simulink model "Copy_of_sistema"  (R2026b)
settings: Solver=VariableStepAuto  MaxStep=1e-3
libraries: slpidlib x1
settings Model: LastModifiedBy=Emiliano
settings DataIOCC: DSMLogging=off  ReturnWorkspaceOutputs=off  SaveOutput=off  SignalLogging=off  TimeSaveName=t
settings DebuggingCC: AlgebraicLoopMsg=none  ArtificialAlgebraicLoopMsg=none  MaxConsecutiveZCsMsg=none

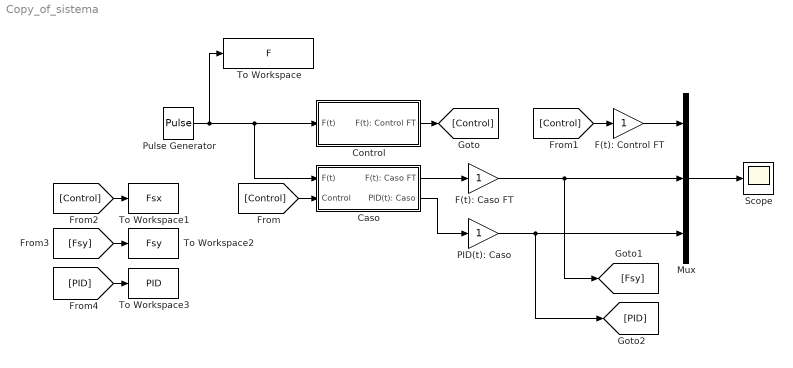
== system Copy_of_sistema ==
  Caso : Subsystem
  Control : Subsystem
  F(t): Caso FT : Gain
  F(t): Control FT : Gain
  Mux : Mux  Inputs=3
  PID(t): Caso : Gain
  Pulse Generator : DiscretePulseGenerator  PulseType=Time based  Period=10  PulseWidth=10  PhaseDelay=1
  Scope : Scope
      settings: ActiveDisplayYMinimum=-0.2  ActiveDisplayYMaximum=1
  To Workspace : ToWorkspace  VariableName=F  SampleTime=-1
  To Workspace1 : ToWorkspace  VariableName=Fsx  SampleTime=-1
  To Workspace2 : ToWorkspace  VariableName=Fsy  SampleTime=-1
  To Workspace3 : ToWorkspace  VariableName=PID  SampleTime=-1
  wires:
  Pulse Generator/1 -> To Workspace/1, Caso/1(F(t)), Control/1(F(t))
  Mux/1 -> Scope/1
  Control/1(F(t): Control FT) -> [Control]
  [Control] -> Caso/2(Control)
  Caso/1(F(t): Caso FT) -> F(t): Caso FT/1
  F(t): Caso FT/1 -> [Fsy], Mux/2
  Caso/2(PID(t): Caso) -> PID(t): Caso/1
  PID(t): Caso/1 -> [PID], Mux/3
  [Control] -> F(t): Control FT/1
  F(t): Control FT/1 -> Mux/1
  [Control] -> To Workspace1/1
  [Fsy] -> To Workspace2/1
  [PID] -> To Workspace3/1

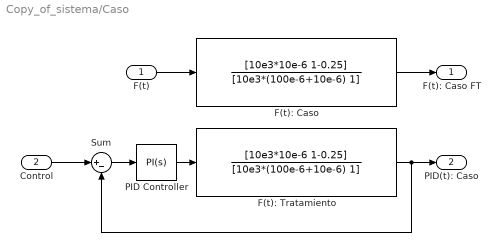
== system Copy_of_sistema/Caso ==
  F(t) : Inport
  Control : Inport  Port=2
  F(t): Caso : TransferFcn  Numerator=[10e3*10e-6 1-0.25]  Denominator=[10e3*(100e-6+10e-6) 1]
  F(t): Tratamiento : TransferFcn  Numerator=[10e3*10e-6 1-0.25]  Denominator=[10e3*(100e-6+10e-6) 1]
  PID Controller : slpidlib/PID Controller  Controller=PI  Form=Parallel  TimeDomain=Continuous-time  UseExternalTs=off  SampleTime=-1  IntegratorMethod=Forward Euler  FilterMethod=Forward Euler  ControllerParametersSource=internal  P=0.019136  I=47422.9366  UseKiTs=off  D=0  UseExternalDerivativeSource=off  N=100  UseFilter=on  TunerSelectOption=Transfer Function Based (PID Tuner App)  InitialConditionSource=internal  InitialConditionForIntegrator=0  InitialConditionForFilter=0  DifferentiatorICPrevScaledInput=0  ExternalReset=none  TrackingMode=off  Kt=1  LimitOutput=off  SatLimitsSource=internal  UpperSaturationLimit=inf  LowerSaturationLimit=-inf  LinearizeAsGain=on  AntiWindupMode=none  Kb=1  LimitIntegrator=off  UpperIntegratorSaturationLimit=inf  LowerIntegratorSaturationLimit=-inf  POutMin=[]  POutMax=[]  IOutMin=[]  IOutMax=[]  DOutMin=[]  DOutMax=[]  NOutMin=[]  NOutMax=[]  SumOutMin=[]  SumOutMax=[]  SaturationOutMin=[]  SaturationOutMax=[]  PParamMin=[]  PParamMax=[]  IParamMin=[]  IParamMax=[]  DParamMin=[]  DParamMax=[]  NParamMin=[]  NParamMax=[]  KbParamMin=[]  KbParamMax=[]  KtParamMin=[]  KtParamMax=[]  KbOutMin=[]  KbOutMax=[]  KtOutMin=[]  KtOutMax=[]  IntegratorOutMin=[]  IntegratorOutMax=[]  FilterOutMin=[]  FilterOutMax=[]  SumI1OutMin=[]  SumI1OutMax=[]  SumI2OutMin=[]  SumI2OutMax=[]  SumI3OutMin=[]  SumI3OutMax=[]  SumI4OutMin=[]  SumI4OutMax=[]  SumDOutMin=[]  SumDOutMax=[]  DifferentiatorOutMin=[]  DifferentiatorOutMax=[]  FilterDiffOutCoefMin=[]  FilterDiffOutCoefMax=[]  ReciprocalOutMin=[]  ReciprocalOutMax=[]  SumDenOutMin=[]  SumDenOutMax=[]  SumNumOutMin=[]  SumNumOutMax=[]  DivideOutMin=[]  DivideOutMax=[]  UdiffTsProdOutMin=[]  UdiffTsProdOutMax=[]  NTsProdOutMin=[]  NTsProdOutMax=[]  UintegralTsProdOutMin=[]  UintegralTsProdOutMax=[]  UngainTsProdOutMin=[]  UngainTsProdOutMax=[]  ClampingZeroOutDataTypeStr=Inherit: Inherit via back propagation  ClampingZeroOutMin=[]  ClampingZeroOutMax=[]  FilterDenConstantOutDataTypeStr=Inherit: Inherit via back propagation  FilterDenConstantOutMin=[]  FilterDenConstantOutMax=[]  PCopyOutDataTypeStr=Inherit: Inherit via back propagation  PCopyOutMin=[]  PCopyOutMax=[]  NCopyOutDataTypeStr=Inherit: Inherit via back propagation  NCopyOutMin=[]  NCopyOutMax=[]  IntegratorContinuousStateAttributes=''  IntegratorStateMustResolveToSignalObject=off  IntegratorRTWStateStorageClass=Auto  FilterContinuousStateAttributes=''  FilterStateMustResolveToSignalObject=off  FilterRTWStateStorageClass=Auto  ParallelPVariant=InternalParameters  IdealPVariant=Disabled  IVariant=InternalParameters  DVariant=Disabled  IntegratorVariant=Continuous  SatVariant=Disabled  AWVariant=Passthrough  PCopyVariant=Disabled  TRVariant=Disabled  FdbkBlocksVariant=Forward  IdealPFdbkVariant=Disabled  SatFdbkVariant=Disabled  DerivativeFilterVariant=Disabled  NVariant=Disabled  NCopyVariant=Disabled_SignalSpec  FilterICVariant=Disabled  IntegratorICVariant=InternalICs  ExternalResetVariant=Disabled  TRSumVariant=Passthrough  SumFdbkVariant=Disabled  SumVariant=Sum_PI  TsampFilterVariant=InternalTs  TsampNgainVariant=Passthrough  TsampIntegralVariant=Disabled_SignalSpec  ExternalSaturationOutDataTypeStr=Inherit: Same as second input  DerivativeSourceVariant=Disabled  PreIntVariant=InternalPreInt
  Sum : Sum  Inputs=|+-
  F(t): Caso FT : Outport
  PID(t): Caso : Outport  Port=2
  wires:
  F(t)/1 -> F(t): Caso/1
  F(t): Caso/1 -> F(t): Caso FT/1
  F(t): Tratamiento/1 -> PID(t): Caso/1, Sum/2
  Control/1 -> Sum/1
  PID Controller/1 -> F(t): Tratamiento/1
  Sum/1 -> PID Controller/1

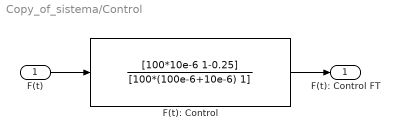
== system Copy_of_sistema/Control ==
  F(t) : Inport
  F(t): Control : TransferFcn  Numerator=[100*10e-6 1-0.25]  Denominator=[100*(100e-6+10e-6) 1]
  F(t): Control FT : Outport
  wires:
  F(t)/1 -> F(t): Control/1
  F(t): Control/1 -> F(t): Control FT/1
